simulink model "Termico_FP"  (R2026b)
settings: Solver=ode45  StopTime=N-1  RelTol=1e-8  EnableMultiTasking=on
values from neighbouring files (symbols this model uses):
  Ct = 0.0002    [Termico_FP_dados.m]
  Ka = 1    [Termico_FP_dados.m]
  Kp = 0.1239    [Termico_FP_dados.m]    (also in estimar_p2dz.m = sys_p2dz.Kp)
  Kt = 9.1657    [Termico_FP_dados.m]
  Kw = 4    [Termico_FP_dados.m]
  Ta = 23.5    [Termico_FP_dados.m]    (also in ma31500.mat = 23.6669092063; preparar_dados.m = mean(Ta_raw))
  Td = 6.67    [Termico_FP_dados.m]    (also in estimar_p2dz.m = sys_p2dz.Td)
  Tp1 = 449.04    [Termico_FP_dados.m]    (also in estimar_p2dz.m = sys_p2dz.Tp1)
  Tp2 = 31.96    [Termico_FP_dados.m]    (also in estimar_p2dz.m = sys_p2dz.Tp2)
  Ts = Td / 2    (= 3.335)    [Termico_FP_dados.m]    (also in estimar_p2dz.m = 1; preparar_dados.m = 1)
  Tz = 367.32    [Termico_FP_dados.m]    (also in estimar_p2dz.m = sys_p2dz.Tz)
settings Model: Creator=Adolfo  LastModifiedBy=Andre
settings SolverCC: ZeroCrossControl=DisableAll
settings DataIOCC: LimitDataPoints=on  MaxDataPoints=25000  ReturnWorkspaceOutputs=off  SaveFormat=Array  SignalLoggingSaveFormat=ModelDataLogs
settings OptimizationCC: BlockReduction=off  BooleanDataType=off  LifeSpan=inf  MemsetInitFltsAndDblsToZero=off  ReuseModelBlockBuffer=off
settings DebuggingCC: ArithmeticOperatorsInVariantConditions=warning  FcnCallInpInsideContextMsg=warning  MergeDetectMultiDrivingBlocksExec=none  MultiTaskCondExecSysMsg=none  MultiTaskDSMMsg=warning  SFExecutionAtInitializationDiag=none  SFNoUnconditionalDefaultTransitionDiag=warning  SFUnexpectedBacktrackingDiag=warning  SaveWithParameterizedLinksMsg=none  SignalResolutionControl=TryResolveAllWithWarning  StateNameClashWarn=warning  UnderspecifiedInitializationDetection=Classic
settings HardwareCC: ProdEndianess=Unspecified  ProdHWDeviceType=32-bit Generic  ProdIntDivRoundTo=Undefined  ProdLargestAtomicFloat=None  TargetUnknown=on
settings ModelReferenceCC: PropagateSignalLabelsOutOfModel=off
settings SFSimCC: CustomCodeUndefinedFunction=UseInterfaceOnly  SimUseLocalCustomCode=off
settings RTWCC: RTWUseLocalCustomCode=off
settings CodeAppCC: StateflowObjectComments=on
settings GRTTargetCC: CombineOutputUpdateFcns=off  GRTInterface=on  TargetFcnLib=ansi_tfl_tmw.mat  TargetLangStandard=C89/C90 (ANSI)
settings ConfigComp: CovExternalEMLEnable=off  CovSaveCumulativeToWorkspaceVar=on  CovSaveSingleToWorkspaceVar=on

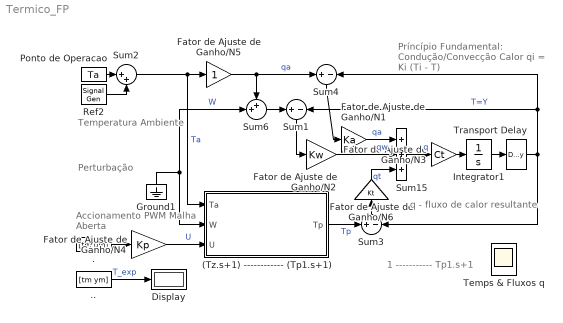
== system Termico_FP ==
  note: Accionamento
      | PWM
      | Malha Aberta
  note: Perturbação
  note: Príncípio Fundamental:
      | Condução/Convecção Calor
      |
      |              qi = Ki (Ti - T)
  note: 1
      |  -----------
      |  Tp1.s+1
  note: q - fluxo de
      | calor resultante
  note: Temperatura Ambiente
  (Tz.s+1) ------------ (Tp1.s+1) : Subsystem
  . : FromWorkspace  VariableName=[tm um]  SampleTime=Ts
  .. : FromWorkspace  VariableName=[tm ym]  SampleTime=Ts
  Display : Display
  Fator de Ajuste de Ganho/N1 : Gain  Gain=Ka  SaturateOnIntegerOverflow=on  OutDataTypeStr=Inherit: Same as input  ParamDataTypeStr=Inherit: Same as input
  Fator de Ajuste de Ganho/N2 : Gain  Gain=Kw  SaturateOnIntegerOverflow=on  OutDataTypeStr=Inherit: Same as input  ParamDataTypeStr=Inherit: Same as input
  Fator de Ajuste de Ganho/N3 : Gain  Gain=Ct  SaturateOnIntegerOverflow=on  OutDataTypeStr=Inherit: Same as input  ParamDataTypeStr=Inherit: Same as input
  Fator de Ajuste de Ganho/N4 : Gain  Gain=Kp  SaturateOnIntegerOverflow=on  OutDataTypeStr=Inherit: Same as input  ParamDataTypeStr=Inherit: Same as input
  Fator de Ajuste de Ganho/N5 : Gain  SaturateOnIntegerOverflow=on  OutDataTypeStr=Inherit: Same as input  ParamDataTypeStr=Inherit: Same as input
  Fator de Ajuste de Ganho/N6 : Gain  Gain=Kt  SaturateOnIntegerOverflow=on  OutDataTypeStr=Inherit: Same as input  ParamDataTypeStr=Inherit: Same as input
  Ground1 : Ground
  Integrator1 : Integrator  InitialCondition=Ta
  Ponto de Operacao : Constant  Value=Ta
  Ref2 : SignalGenerator  Amplitude=2  Frequency=1/3600/24
  Sum1 : Sum  Inputs=+|-  InputSameDT=on  SaturateOnIntegerOverflow=on  OutDataTypeStr=Inherit: Same as first input
  Sum15 : Sum  Inputs=+++  InputSameDT=on  SaturateOnIntegerOverflow=on  OutDataTypeStr=Inherit: Same as first input
  Sum2 : Sum  Inputs=|++
  Sum3 : Sum  Inputs=+|-  InputSameDT=on  SaturateOnIntegerOverflow=on  OutDataTypeStr=Inherit: Same as first input
  Sum4 : Sum  Inputs=+|-  InputSameDT=on  SaturateOnIntegerOverflow=on  OutDataTypeStr=Inherit: Same as first input
  Sum6 : Sum  Inputs=++|
  Temps & Fluxos q : Scope
      settings: IsFloating=on  Floating=on  TimeSpan=N-1  ActiveDisplayYMinimum=10.06402  ActiveDisplayYMaximum=57.14462
  Transport Delay : TransportDelay  DelayTime=Td  InitialOutput=Ta  BufferSize=2048  PadeOrder=2
  wires:
  Sum15/1 -> Fator de Ajuste de Ganho/N3/1  "q"
  Fator de Ajuste de Ganho/N3/1 -> Integrator1/1
  Sum3/1 -> Fator de Ajuste de Ganho/N6/1
  Fator de Ajuste de Ganho/N4/1 -> (Tz.s+1) ------------ (Tp1.s+1)/3(U)  "U"
  Transport Delay/1 -> Sum3/2, Sum1/2, Sum4/2  "T=Y"
  (Tz.s+1) ------------ (Tp1.s+1)/1(Tp) -> Sum3/1  "Tp"
  Fator de Ajuste de Ganho/N6/1 -> Sum15/3  "qt"
  Ponto de Operacao/1 -> Sum2/1
  Sum1/1 -> Fator de Ajuste de Ganho/N2/1
  Integrator1/1 -> Transport Delay/1
  Ground1/1 -> (Tz.s+1) ------------ (Tp1.s+1)/2(W), Sum6/2  "W"
  Fator de Ajuste de Ganho/N2/1 -> Sum15/2  "qw"
  ./1 -> Fator de Ajuste de Ganho/N4/1
  Sum4/1 -> Fator de Ajuste de Ganho/N1/1
  Fator de Ajuste de Ganho/N1/1 -> Sum15/1  "qa"
  Sum6/1 -> Sum1/1
  ../1 -> Display/1  "T_exp"
  Ref2/1 -> Sum2/2
  Sum2/1 -> Fator de Ajuste de Ganho/N5/1, (Tz.s+1) ------------ (Tp1.s+1)/1(Ta)  "Ta"
  Fator de Ajuste de Ganho/N5/1 -> Sum6/1, Sum4/1  "qa"

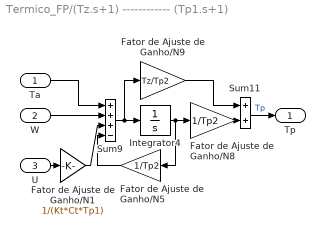
== system Termico_FP/(Tz.s+1) ------------ (Tp1.s+1) ==
  Ta : Inport
  W : Inport  Port=2
  U : Inport  Port=3
  Fator de Ajuste de Ganho/N1 : Gain  Gain=1/(Kt*Ct*Tp1)  SaturateOnIntegerOverflow=on  OutDataTypeStr=Inherit: Same as input  ParamDataTypeStr=Inherit: Same as input
  Fator de Ajuste de Ganho/N5 : Gain  Gain=1/Tp2  SaturateOnIntegerOverflow=on  OutDataTypeStr=Inherit: Same as input  ParamDataTypeStr=Inherit: Same as input
  Fator de Ajuste de Ganho/N8 : Gain  Gain=1/Tp2  SaturateOnIntegerOverflow=on  OutDataTypeStr=Inherit: Same as input  ParamDataTypeStr=Inherit: Same as input
  Fator de Ajuste de Ganho/N9 : Gain  Gain=Tz/Tp2  SaturateOnIntegerOverflow=on  OutDataTypeStr=Inherit: Same as input  ParamDataTypeStr=Inherit: Same as input
  Integrator4 : Integrator  InitialCondition=Ta*Tp2
  Sum11 : Sum  InputSameDT=on  SaturateOnIntegerOverflow=on  OutDataTypeStr=Inherit: Same as first input
  Sum9 : Sum  Inputs=+++-
  Tp : Outport
  wires:
  Ta/1 -> Sum9/1
  Fator de Ajuste de Ganho/N5/1 -> Sum9/4
  Sum11/1 -> Tp/1  "Tp"
  U/1 -> Fator de Ajuste de Ganho/N1/1
  Fator de Ajuste de Ganho/N9/1 -> Sum11/1
  Fator de Ajuste de Ganho/N8/1 -> Sum11/2
  W/1 -> Sum9/2
  Sum9/1 -> Fator de Ajuste de Ganho/N9/1, Integrator4/1
  Integrator4/1 -> Fator de Ajuste de Ganho/N8/1, Fator de Ajuste de Ganho/N5/1
  Fator de Ajuste de Ganho/N1/1 -> Sum9/3
